simulink model "p1_2_ecc"  (R2025b)
settings: Solver=ode45  StartTime=0.0  StopTime=1  MaxStep=1e-3  RelTol=1e-6
undefined symbols (not defined in the file or in its folder): mp
settings Model: Creator=maria  LastModifiedBy=maria

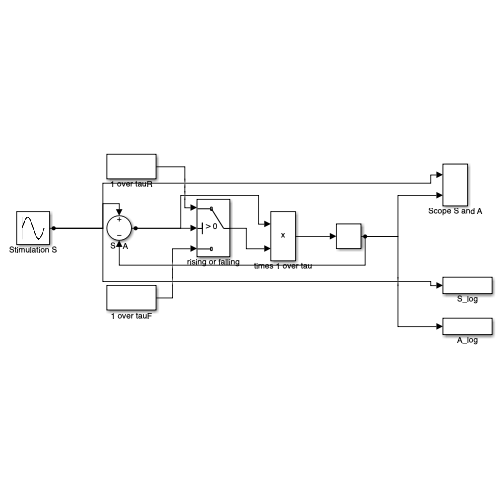
[thumbnail: Simulink's stored preview of the top-level diagram]
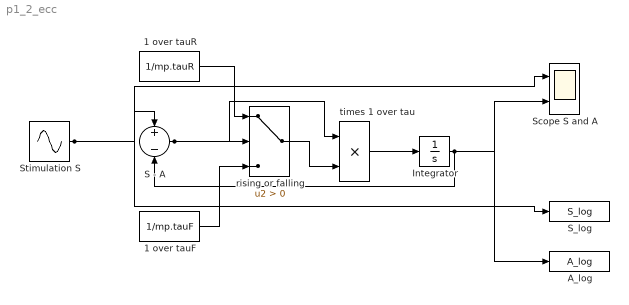
== system p1_2_ecc ==
  1 over tauF : Constant  Value=1/mp.tauF
  1 over tauR : Constant  Value=1/mp.tauR
  A_log : ToWorkspace  VariableName=A_log  SaveFormat=Timeseries  SampleTime=-1
  Integrator : Integrator  InitialCondition=mp.A0
  S - A : Sum  Inputs=+-
  S_log : ToWorkspace  VariableName=S_log  SaveFormat=Timeseries  SampleTime=-1
  Scope S and A : Scope  NumInputPorts=2
  Stimulation S : Sin  Amplitude=0.5  Bias=0.5  Frequency=2*pi  SampleTime=0
  rising or falling : Switch  Criteria=u2 > Threshold  SaturateOnIntegerOverflow=off  InputSameDT=off
  times 1 over tau : Product
  wires:
  Stimulation S/1 -> S - A/1, Scope S and A/1, S_log/1
  S - A/1 -> rising or falling/2, times 1 over tau/1
  1 over tauR/1 -> rising or falling/1
  1 over tauF/1 -> rising or falling/3
  rising or falling/1 -> times 1 over tau/2
  times 1 over tau/1 -> Integrator/1
  Integrator/1 -> S - A/2, Scope S and A/2, A_log/1
